simulink model "PCProject3"  (R2024a)
settings: Solver=VariableStepAuto  StartTime=0.0  StopTime=50.0  RelTol=1e-3
(part 1 of 7)
settings Model: Creator=User  LastModifiedBy=User

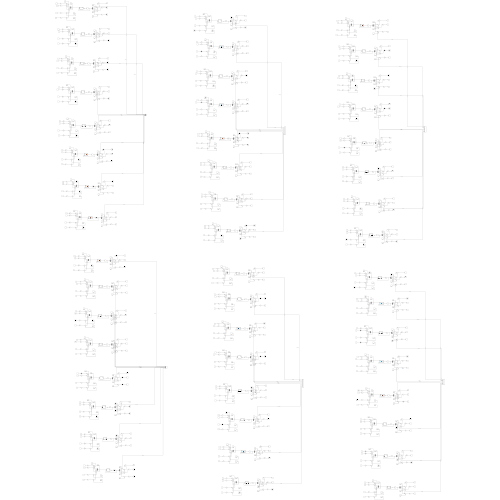
[thumbnail: Simulink's stored preview of the top-level diagram]
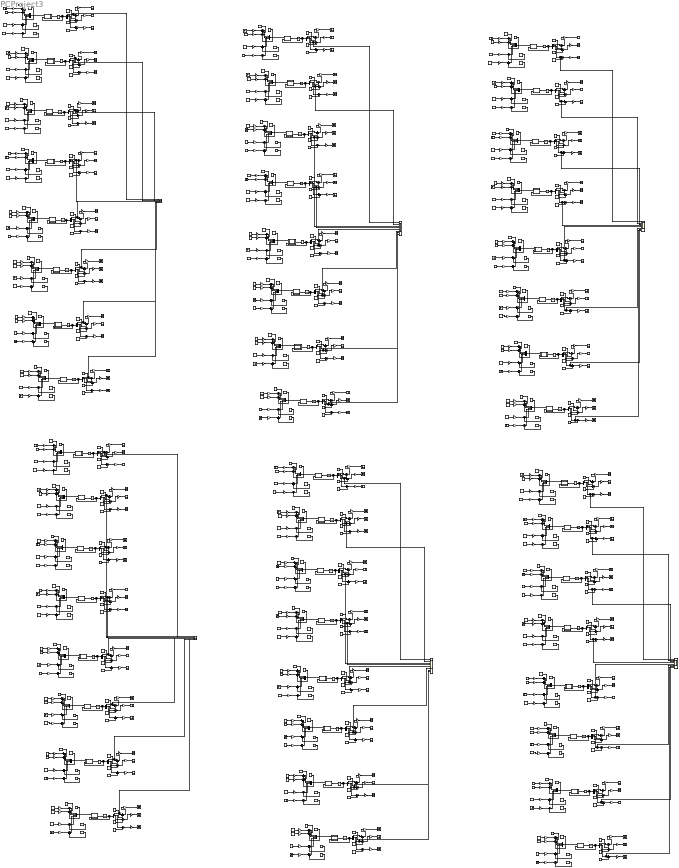
== system PCProject3 ==
  Bss{,1..47} (48 alike) : Constant  Value=9.44585785232475
  Constant{1..144} (144 alike) : Constant  Value=0
  Demux{,1..47} (48 alike) : Demux  Outputs=7
  F0ss{,1..47} (48 alike) : Constant  Value=100
  F_PUss{,1..47} (48 alike) : Constant  Value=25
  F_css{,1..47} (48 alike) : Constant  Value=500
  Gain{,7,14,21,28,35,42,49,56,62,70,77,85,93,100,109,112,118,126,133,141,149,156,165,168,171,180,184,190,199,207,214,216,224,232,242,250,257,265,273,280,288,295,303..304,311,320,329} (48 alike) : Gain  Gain=142.9/100
  Gain{1,8,15,22,29,36,43,50,57,63,71,78,86,94,102,110,113,119,127,134,142,150,158,166,169,173,182,185,191,200,208,217,225..226,234,243,251,258,266,274,282,289,296,305,312,314,321,330} (48 alike) : Gain  Gain=500/100
  Gain{3,10,17,24,31,38,45,52,58,65,73,79,81,88,96,104,114,121,129,135,137,144,152,160,170,175,186,194,202,209,211,219,228,237,245,253,259,261,268,276,284,290,298,307,313,316,323,332} (48 alike) : Gain  Gain=100/100
  Gain{5,12,19,26,33,40,46,54,60,67,75,83,91,98,101,106,116,123,131,139,147,154,157,162,172,177,188,192,196,205,213,222,230,233,239,247,255,263,271,278,281,286,293,300,309,318,327,334} (48 alike) : Gain  Gain=100/61.6246329506498
  Gain{2,9,16,23,30,37,44,51,64,68,72,80,87,95,103,111,120,124,128,136,143,151,159,167,174,183,193,197,201,210,218,227,235..236,244,248,252,260,267,275,283,297,301,306,315,322,325,331} (48 alike) : Gain  Gain=25/100
  Gain{4,11,18,25,32,39,53,59,66,74,82,89..90,97,105,115,122,130,138,145..146,153,161,176,181,187,195,204,212,220..221,229,238,246,254,262,269..270,277,285,291,299,308,317,324,326,333,336} (48 alike) : Gain  Gain=100/21.5066564396397
  Gain{6,13,20,27,34,41,47,55,61,69,76,84,92,99,107..108,117,125,132,140,148,155,163..164,178..179,189,198,203,206,215,223,231,240..241,249,256,264,272,279,287,292,294,302,310,319,328,335} (48 alike) : Gain  Gain=100/9.44585785232475
  Integrator : Integrator  InitialCondition=|
      | [21.5066564396397
      | 61.6246329506498
      | 9.44585785232475
      | 2.44473177554800
      | 0.491745288474893
      | 3.01943696537133
      | 2.73422289591667]
  Integrator1 : Integrator  InitialCondition=|
      | [21.5066564396397
      | 61.6246329506498
      | 9.44585785232475
      | 2.44473177554800
      | 0.491745288474893
      | 3.01943696537133
      | 2.73422289591667]
  Integrator10 : Integrator  InitialCondition=|
      | [21.5066564396397
      | 61.6246329506498
      | 9.44585785232475
      | 2.44473177554800
      | 0.491745288474893
      | 3.01943696537133
      | 2.73422289591667]
  Integrator11 : Integrator  InitialCondition=|
      | [21.5066564396397
      | 61.6246329506498
      | 9.44585785232475
      | 2.44473177554800
      | 0.491745288474893
      | 3.01943696537133
      | 2.73422289591667]
  Integrator12 : Integrator  InitialCondition=|
      | [21.5066564396397
      | 61.6246329506498
      | 9.44585785232475
      | 2.44473177554800
      | 0.491745288474893
      | 3.01943696537133
      | 2.73422289591667]
  Integrator13 : Integrator  InitialCondition=|
      | [21.5066564396397
      | 61.6246329506498
      | 9.44585785232475
      | 2.44473177554800
      | 0.491745288474893
      | 3.01943696537133
      | 2.73422289591667]
  Integrator14 : Integrator  InitialCondition=|
      | [21.5066564396397
      | 61.6246329506498
      | 9.44585785232475
      | 2.44473177554800
      | 0.491745288474893
      | 3.01943696537133
      | 2.73422289591667]
  Integrator15 : Integrator  InitialCondition=|
      | [21.5066564396397
      | 61.6246329506498
      | 9.44585785232475
      | 2.44473177554800
      | 0.491745288474893
      | 3.01943696537133
      | 2.73422289591667]
  Integrator16 : Integrator  InitialCondition=|
      | [21.5066564396397
      | 61.6246329506498
      | 9.44585785232475
      | 2.44473177554800
      | 0.491745288474893
      | 3.01943696537133
      | 2.73422289591667]
  Integrator17 : Integrator  InitialCondition=|
      | [21.5066564396397
      | 61.6246329506498
      | 9.44585785232475
      | 2.44473177554800
      | 0.491745288474893
      | 3.01943696537133
      | 2.73422289591667]
  Integrator18 : Integrator  InitialCondition=|
      | [21.5066564396397
      | 61.6246329506498
      | 9.44585785232475
      | 2.44473177554800
      | 0.491745288474893
      | 3.01943696537133
      | 2.73422289591667]
  Integrator19 : Integrator  InitialCondition=|
      | [21.5066564396397
      | 61.6246329506498
      | 9.44585785232475
      | 2.44473177554800
      | 0.491745288474893
      | 3.01943696537133
      | 2.73422289591667]
  Integrator2 : Integrator  InitialCondition=|
      | [21.5066564396397
      | 61.6246329506498
      | 9.44585785232475
      | 2.44473177554800
      | 0.491745288474893
      | 3.01943696537133
      | 2.73422289591667]
  Integrator20 : Integrator  InitialCondition=|
      | [21.5066564396397
      | 61.6246329506498
      | 9.44585785232475
      | 2.44473177554800
      | 0.491745288474893
      | 3.01943696537133
      | 2.73422289591667]
  Integrator21 : Integrator  InitialCondition=|
      | [21.5066564396397
      | 61.6246329506498
      | 9.44585785232475
      | 2.44473177554800
      | 0.491745288474893
      | 3.01943696537133
      | 2.73422289591667]
  Integrator22 : Integrator  InitialCondition=|
      | [21.5066564396397
      | 61.6246329506498
      | 9.44585785232475
      | 2.44473177554800
      | 0.491745288474893
      | 3.01943696537133
      | 2.73422289591667]
  Integrator23 : Integrator  InitialCondition=|
      | [21.5066564396397
      | 61.6246329506498
      | 9.44585785232475
      | 2.44473177554800
      | 0.491745288474893
      | 3.01943696537133
      | 2.73422289591667]
  Integrator24 : Integrator  InitialCondition=|
      | [21.5066564396397
      | 61.6246329506498
      | 9.44585785232475
      | 2.44473177554800
      | 0.491745288474893
      | 3.01943696537133
      | 2.73422289591667]
  Integrator25 : Integrator  InitialCondition=|
      | [21.5066564396397
      | 61.6246329506498
      | 9.44585785232475
      | 2.44473177554800
      | 0.491745288474893
      | 3.01943696537133
      | 2.73422289591667]
  Integrator26 : Integrator  InitialCondition=|
      | [21.5066564396397
      | 61.6246329506498
      | 9.44585785232475
      | 2.44473177554800
      | 0.491745288474893
      | 3.01943696537133
      | 2.73422289591667]
  Integrator27 : Integrator  InitialCondition=|
      | [21.5066564396397
      | 61.6246329506498
      | 9.44585785232475
      | 2.44473177554800
      | 0.491745288474893
      | 3.01943696537133
      | 2.73422289591667]
  Integrator28 : Integrator  InitialCondition=|
      | [21.5066564396397
      | 61.6246329506498
      | 9.44585785232475
      | 2.44473177554800
      | 0.491745288474893
      | 3.01943696537133
      | 2.73422289591667]
  Integrator29 : Integrator  InitialCondition=|
      | [21.5066564396397
      | 61.6246329506498
      | 9.44585785232475
      | 2.44473177554800
      | 0.491745288474893
      | 3.01943696537133
      | 2.73422289591667]
  Integrator3 : Integrator  InitialCondition=|
      | [21.5066564396397
      | 61.6246329506498
      | 9.44585785232475
      | 2.44473177554800
      | 0.491745288474893
      | 3.01943696537133
      | 2.73422289591667]
  Integrator30 : Integrator  InitialCondition=|
      | [21.5066564396397
      | 61.6246329506498
      | 9.44585785232475
      | 2.44473177554800
      | 0.491745288474893
      | 3.01943696537133
      | 2.73422289591667]
  Integrator31 : Integrator  InitialCondition=|
      | [21.5066564396397
      | 61.6246329506498
      | 9.44585785232475
      | 2.44473177554800
      | 0.491745288474893
      | 3.01943696537133
      | 2.73422289591667]
  Integrator32 : Integrator  InitialCondition=|
      | [21.5066564396397
      | 61.6246329506498
      | 9.44585785232475
      | 2.44473177554800
      | 0.491745288474893
      | 3.01943696537133
      | 2.73422289591667]
  Integrator33 : Integrator  InitialCondition=|
      | [21.5066564396397
      | 61.6246329506498
      | 9.44585785232475
      | 2.44473177554800
      | 0.491745288474893
      | 3.01943696537133
      | 2.73422289591667]
  Integrator34 : Integrator  InitialCondition=|
      | [21.5066564396397
      | 61.6246329506498
      | 9.44585785232475
      | 2.44473177554800
      | 0.491745288474893
      | 3.01943696537133
      | 2.73422289591667]
  Integrator35 : Integrator  InitialCondition=|
      | [21.5066564396397
      | 61.6246329506498
      | 9.44585785232475
      | 2.44473177554800
      | 0.491745288474893
      | 3.01943696537133
      | 2.73422289591667]
  Integrator36 : Integrator  InitialCondition=|
      | [21.5066564396397
      | 61.6246329506498
      | 9.44585785232475
      | 2.44473177554800
      | 0.491745288474893
      | 3.01943696537133
      | 2.73422289591667]
  Integrator37 : Integrator  InitialCondition=|
      | [21.5066564396397
      | 61.6246329506498
      | 9.44585785232475
      | 2.44473177554800
      | 0.491745288474893
      | 3.01943696537133
      | 2.73422289591667]
  Integrator38 : Integrator  InitialCondition=|
      | [21.5066564396397
      | 61.6246329506498
      | 9.44585785232475
      | 2.44473177554800
      | 0.491745288474893
      | 3.01943696537133
      | 2.73422289591667]
  Integrator39 : Integrator  InitialCondition=|
      | [21.5066564396397
      | 61.6246329506498
      | 9.44585785232475
      | 2.44473177554800
      | 0.491745288474893
      | 3.01943696537133
      | 2.73422289591667]
  Integrator4 : Integrator  InitialCondition=|
      | [21.5066564396397
      | 61.6246329506498
      | 9.44585785232475
      | 2.44473177554800
      | 0.491745288474893
      | 3.01943696537133
      | 2.73422289591667]
  Integrator40 : Integrator  InitialCondition=|
      | [21.5066564396397
      | 61.6246329506498
      | 9.44585785232475
      | 2.44473177554800
      | 0.491745288474893
      | 3.01943696537133
      | 2.73422289591667]
  Integrator41 : Integrator  InitialCondition=|
      | [21.5066564396397
      | 61.6246329506498
      | 9.44585785232475
      | 2.44473177554800
      | 0.491745288474893
      | 3.01943696537133
      | 2.73422289591667]
  Integrator42 : Integrator  InitialCondition=|
      | [21.5066564396397
      | 61.6246329506498
      | 9.44585785232475
      | 2.44473177554800
      | 0.491745288474893
      | 3.01943696537133
      | 2.73422289591667]
  Integrator43 : Integrator  InitialCondition=|
      | [21.5066564396397
      | 61.6246329506498
      | 9.44585785232475
      | 2.44473177554800
      | 0.491745288474893
      | 3.01943696537133
      | 2.73422289591667]
  Integrator44 : Integrator  InitialCondition=|
      | [21.5066564396397
      | 61.6246329506498
      | 9.44585785232475
      | 2.44473177554800
      | 0.491745288474893
      | 3.01943696537133
      | 2.73422289591667]
  Integrator45 : Integrator  InitialCondition=|
      | [21.5066564396397
      | 61.6246329506498
      | 9.44585785232475
      | 2.44473177554800
      | 0.491745288474893
      | 3.01943696537133
      | 2.73422289591667]
  Integrator46 : Integrator  InitialCondition=|
      | [21.5066564396397
      | 61.6246329506498
      | 9.44585785232475
      | 2.44473177554800
      | 0.491745288474893
      | 3.01943696537133
      | 2.73422289591667]
  Integrator47 : Integrator  InitialCondition=|
      | [21.5066564396397
      | 61.6246329506498
      | 9.44585785232475
      | 2.44473177554800
      | 0.491745288474893
      | 3.01943696537133
      | 2.73422289591667]
  Integrator5 : Integrator  InitialCondition=|
      | [21.5066564396397
      | 61.6246329506498
      | 9.44585785232475
      | 2.44473177554800
      | 0.491745288474893
      | 3.01943696537133
      | 2.73422289591667]
  Integrator6 : Integrator  InitialCondition=|
      | [21.5066564396397
      | 61.6246329506498
      | 9.44585785232475
      | 2.44473177554800
      | 0.491745288474893
      | 3.01943696537133
      | 2.73422289591667]
  Integrator7 : Integrator  InitialCondition=|
      | [21.5066564396397
      | 61.6246329506498
      | 9.44585785232475
      | 2.44473177554800
      | 0.491745288474893
      | 3.01943696537133
      | 2.73422289591667]
  Integrator8 : Integrator  InitialCondition=|
      | [21.5066564396397
      | 61.6246329506498
      | 9.44585785232475
      | 2.44473177554800
      | 0.491745288474893
      | 3.01943696537133
      | 2.73422289591667]
  Integrator9 : Integrator  InitialCondition=|
      | [21.5066564396397
      | 61.6246329506498
      | 9.44585785232475
      | 2.44473177554800
      | 0.491745288474893
      | 3.01943696537133
      | 2.73422289591667]
  MATLAB Function : MATLAB Function  TreatAsAtomicUnit=on
  MATLAB Function1 : MATLAB Function  TreatAsAtomicUnit=on
  MATLAB Function10 : MATLAB Function  TreatAsAtomicUnit=on
  MATLAB Function11 : MATLAB Function  TreatAsAtomicUnit=on
  MATLAB Function12 : MATLAB Function  TreatAsAtomicUnit=on
  MATLAB Function13 : MATLAB Function  TreatAsAtomicUnit=on
  MATLAB Function14 : MATLAB Function  TreatAsAtomicUnit=on
  MATLAB Function15 : MATLAB Function  TreatAsAtomicUnit=on
  MATLAB Function16 : MATLAB Function  TreatAsAtomicUnit=on
  MATLAB Function17 : MATLAB Function  TreatAsAtomicUnit=on
  MATLAB Function18 : MATLAB Function  TreatAsAtomicUnit=on
  MATLAB Function19 : MATLAB Function  TreatAsAtomicUnit=on
  MATLAB Function2 : MATLAB Function  TreatAsAtomicUnit=on
  MATLAB Function20 : MATLAB Function  TreatAsAtomicUnit=on
  MATLAB Function21 : MATLAB Function  TreatAsAtomicUnit=on
  MATLAB Function22 : MATLAB Function  TreatAsAtomicUnit=on
  MATLAB Function23 : MATLAB Function  TreatAsAtomicUnit=on
  MATLAB Function24 : MATLAB Function  TreatAsAtomicUnit=on
  MATLAB Function25 : MATLAB Function  TreatAsAtomicUnit=on
  MATLAB Function26 : MATLAB Function  TreatAsAtomicUnit=on
  MATLAB Function27 : MATLAB Function  TreatAsAtomicUnit=on
  MATLAB Function28 : MATLAB Function  TreatAsAtomicUnit=on
  MATLAB Function29 : MATLAB Function  TreatAsAtomicUnit=on
  MATLAB Function3 : MATLAB Function  TreatAsAtomicUnit=on
  MATLAB Function30 : MATLAB Function  TreatAsAtomicUnit=on
  MATLAB Function31 : MATLAB Function  TreatAsAtomicUnit=on
  MATLAB Function32 : MATLAB Function  TreatAsAtomicUnit=on
  MATLAB Function33 : MATLAB Function  TreatAsAtomicUnit=on
  MATLAB Function34 : MATLAB Function  TreatAsAtomicUnit=on
  MATLAB Function35 : MATLAB Function  TreatAsAtomicUnit=on
  MATLAB Function36 : MATLAB Function  TreatAsAtomicUnit=on
  MATLAB Function37 : MATLAB Function  TreatAsAtomicUnit=on
  MATLAB Function38 : MATLAB Function  TreatAsAtomicUnit=on
  MATLAB Function39 : MATLAB Function  TreatAsAtomicUnit=on
  MATLAB Function4 : MATLAB Function  TreatAsAtomicUnit=on
  MATLAB Function40 : MATLAB Function  TreatAsAtomicUnit=on
  MATLAB Function41 : MATLAB Function  TreatAsAtomicUnit=on
  MATLAB Function42 : MATLAB Function  TreatAsAtomicUnit=on
  MATLAB Function43 : MATLAB Function  TreatAsAtomicUnit=on
  MATLAB Function44 : MATLAB Function  TreatAsAtomicUnit=on
  MATLAB Function45 : MATLAB Function  TreatAsAtomicUnit=on
  MATLAB Function46 : MATLAB Function  TreatAsAtomicUnit=on
  MATLAB Function47 : MATLAB Function  TreatAsAtomicUnit=on
  MATLAB Function5 : MATLAB Function  TreatAsAtomicUnit=on
  MATLAB Function6 : MATLAB Function  TreatAsAtomicUnit=on
  MATLAB Function7 : MATLAB Function  TreatAsAtomicUnit=on
  MATLAB Function8 : MATLAB Function  TreatAsAtomicUnit=on
  MATLAB Function9 : MATLAB Function  TreatAsAtomicUnit=on
  Mux{,1..47} (48 alike) : Mux
  S0ss{,1..47} (48 alike) : Constant  Value=142.9
  Scope{,1..2,4..14,16..63,65..74,76..104,106..125,127..149} (144 alike) : Scope
  Scope{3,64,105,150..152} (6 alike) : Scope  NumInputPorts=8
  Sss{,1..47} (48 alike) : Constant  Value=61.6246329506498
  Step{,2,4..5,8,10,12..13,16,18,20..21} (12 alike) : Step  After=5  SampleTime=0
  Step{1,3,6..7,9,11,14..15,17,19,22..23} (12 alike) : Step  After=-5  SampleTime=0
  Step{24,26,28..29,32,34,36..38,42..43,46} (12 alike) : Step  After=30  SampleTime=0
  Step{25,27,30..31,33,35,39..41,44..45,47} (12 alike) : Step  After=-30  SampleTime=0
  Sum{,1..3,7..10,14..17,21..24,28..31,35..38,42..45,49..52,56..58,62..65,68,70..73,77..81,85..88,93..96,100,102..104,109..114,118..121,124,126..129,133..137,141..144,149..152,156,158..160,165..171,173..175,180,182..186,190..191,193..194,197,199..202,207..211,214,216..219,224..228,232,234..237,242..245,248,250..253,257..261,265..268,273..276,280,282..284,288..290,295..298,301,303..307,311..316,320..323,325,329..332} (192 alike) : Sum  Inputs=|++
  Sum{4..6,11..13,18..20,25..27,32..34,39..41,46..48,53..55,59..61,66..67,69,74..76,82..84,89..92,97..99,101,105..108,115..117,122..123,125,130..132,138..140,145..148,153..155,157,161..164,172,176..179,181,187..189,192,195..196,198,203..206,212..213,215,220..223,229..231,233,238..241,246..247,249,254..256,262..264,269..272,277..279,281,285..287,291..294,299..300,302,308..310,317..319,324,326..328,333..335} (144 alike) : Sum  Inputs=|+-
  Xss{,1..47} (48 alike) : Constant  Value=21.5066564396397
  wires:
  Gain2/1 -> Sum2/1
  Step/1 -> Gain/1
  Gain6/1 -> Scope2/1
  Sss/1 -> Sum5/2
  Gain3/1 -> Sum3/1
  Xss/1 -> Sum4/2
  Sum6/1 -> Gain6/1
  F0ss/1 -> Sum3/2
  F_PUss/1 -> Sum2/2
  Sum4/1 -> Gain4/1
  Constant1/1 -> Gain2/1
  Constant2/1 -> Gain1/1
  Bss/1 -> Sum6/2
  Sum5/1 -> Gain5/1
  Integrator/1 -> MATLAB Function/2(x), Demux/1  "x"
  S0ss/1 -> Sum/2
  Gain5/1 -> Scope1/1
  MATLAB Function/1(dxdt) -> Integrator/1  "dxdt"
  Gain4/1 -> Scope/1
  Constant4/1 -> Gain3/1
  Gain1/1 -> Sum1/1
  Mux/1 -> MATLAB Function/1(u)  "u"
  Gain/1 -> Sum/1
  F_css/1 -> Sum1/2
  Sum3/1 -> Mux/1
  Sum2/1 -> Mux/2
  Sum1/1 -> Mux/3
  Sum/1 -> Mux/4
  Demux/1 -> Sum4/1, Scope3/7  "-5% Fc"
  Demux/2 -> Sum5/1
  Demux/3 -> Sum6/1
  Step1/1 -> Gain7/1
  Xss1/1 -> Sum11/2
  MATLAB Function1/1(dxdt) -> Integrator1/1  "dxdt"
  Sum7/1 -> Mux1/4
  Demux1/3 -> Sum13/1
  Demux1/2 -> Sum12/1
  Sum13/1 -> Gain13/1
  Sum12/1 -> Gain12/1
  Constant3/1 -> Gain9/1
  Constant5/1 -> Gain8/1
  Gain9/1 -> Sum9/1
  Gain12/1 -> Scope7/1
  Integrator1/1 -> MATLAB Function1/2(x), Demux1/1  "x"
  Sum8/1 -> Mux1/3
  Gain8/1 -> Sum8/1
  Bss1/1 -> Sum13/2
  Demux1/1 -> Scope3/8, Sum11/1  "-5% S0"
  Sum9/1 -> Mux1/2
  Sum10/1 -> Mux1/1
  F_css1/1 -> Sum8/2
  Mux1/1 -> MATLAB Function1/1(u)  "u"
  Constant6/1 -> Gain10/1
  Gain7/1 -> Sum7/1
  F_PUss1/1 -> Sum9/2
  Gain11/1 -> Scope6/1
  Sum11/1 -> Gain11/1
  Gain13/1 -> Scope8/1
  Sss1/1 -> Sum12/2
  Gain10/1 -> Sum10/1
  F0ss1/1 -> Sum10/2
  S0ss1/1 -> Sum7/2
  Xss2/1 -> Sum18/2
  MATLAB Function2/1(dxdt) -> Integrator2/1  "dxdt"
  Sum14/1 -> Mux2/4
  Demux2/3 -> Sum20/1
  Demux2/2 -> Sum19/1
  Sum20/1 -> Gain20/1
  Sum19/1 -> Gain19/1
  Constant8/1 -> Gain15/1
  Gain16/1 -> Sum16/1
  Gain19/1 -> Scope12/1
  Integrator2/1 -> MATLAB Function2/2(x), Demux2/1  "x"
  Sum15/1 -> Mux2/3
  Gain15/1 -> Sum15/1
  Bss2/1 -> Sum20/2
  Demux2/1 -> Scope3/3, Sum18/1  "+5% Fc"
  Sum16/1 -> Mux2/2
  Sum17/1 -> Mux2/1
  F_css2/1 -> Sum15/2
  Mux2/1 -> MATLAB Function2/1(u)  "u"
  Constant9/1 -> Gain17/1
  Gain14/1 -> Sum14/1
  F_PUss2/1 -> Sum16/2
  Gain18/1 -> Scope11/1
  Sum18/1 -> Gain18/1
  Gain20/1 -> Scope13/1
  Sss2/1 -> Sum19/2
  Gain17/1 -> Sum17/1
  F0ss2/1 -> Sum17/2
  S0ss2/1 -> Sum14/2
  Xss3/1 -> Sum25/2
  MATLAB Function3/1(dxdt) -> Integrator3/1  "dxdt"
  Sum21/1 -> Mux3/4
  Demux3/3 -> Sum27/1
  Demux3/2 -> Sum26/1
  Sum27/1 -> Gain27/1
  Sum26/1 -> Gain26/1
  Constant11/1 -> Gain22/1
  Gain23/1 -> Sum23/1
  Gain26/1 -> Scope17/1
  Integrator3/1 -> MATLAB Function3/2(x), Demux3/1  "x"
  Sum22/1 -> Mux3/3
  Gain22/1 -> Sum22/1
  Bss3/1 -> Sum27/2
  Demux3/1 -> Scope3/4, Sum25/1  "+5% S0"
  Sum23/1 -> Mux3/2
  Sum24/1 -> Mux3/1
  F_css3/1 -> Sum22/2
  Mux3/1 -> MATLAB Function3/1(u)  "u"
  Constant12/1 -> Gain24/1
  Gain21/1 -> Sum21/1
  F_PUss3/1 -> Sum23/2
  Gain25/1 -> Scope16/1
  Sum25/1 -> Gain25/1
  Gain27/1 -> Scope18/1
  Sss3/1 -> Sum26/2
  Gain24/1 -> Sum24/1
  F0ss3/1 -> Sum24/2
  S0ss3/1 -> Sum21/2
  Xss4/1 -> Sum32/2
  MATLAB Function4/1(dxdt) -> Integrator4/1  "dxdt"
  Sum28/1 -> Mux4/4
  Demux4/3 -> Sum34/1
  Demux4/2 -> Sum33/1
  Sum34/1 -> Gain34/1
  Sum33/1 -> Gain33/1
  Constant13/1 -> Gain30/1
  Gain30/1 -> Sum30/1
  Gain33/1 -> Scope22/1
  Integrator4/1 -> MATLAB Function4/2(x), Demux4/1  "x"
  Sum29/1 -> Mux4/3
  Gain29/1 -> Sum29/1
  Bss4/1 -> Sum34/2
  Demux4/1 -> Scope3/5, Sum32/1  "-5% F0"
  Sum30/1 -> Mux4/2
  Sum31/1 -> Mux4/1
  F_css4/1 -> Sum29/2
  Mux4/1 -> MATLAB Function4/1(u)  "u"
  Constant15/1 -> Gain31/1
  Gain28/1 -> Sum28/1
  F_PUss4/1 -> Sum30/2
  Gain32/1 -> Scope21/1
  Sum32/1 -> Gain32/1
  Gain34/1 -> Scope23/1
  Sss4/1 -> Sum33/2
  Gain31/1 -> Sum31/1
  F0ss4/1 -> Sum31/2
  S0ss4/1 -> Sum28/2
  Xss5/1 -> Sum39/2
  MATLAB Function5/1(dxdt) -> Integrator5/1  "dxdt"
  Sum35/1 -> Mux5/4
  Demux5/3 -> Sum41/1
  Demux5/2 -> Sum40/1
  Sum41/1 -> Gain41/1
  Sum40/1 -> Gain40/1
  Constant16/1 -> Gain37/1
  Constant17/1 -> Gain36/1
  Gain37/1 -> Sum37/1
  Gain40/1 -> Scope27/1
  Integrator5/1 -> MATLAB Function5/2(x), Demux5/1  "x"
  Sum36/1 -> Mux5/3
  Gain36/1 -> Sum36/1
  Bss5/1 -> Sum41/2
  Sum37/1 -> Mux5/2
  Sum38/1 -> Mux5/1
  F_css5/1 -> Sum36/2
  Mux5/1 -> MATLAB Function5/1(u)  "u"
  Gain35/1 -> Sum35/1
  F_PUss5/1 -> Sum37/2
  Gain39/1 -> Scope26/1
  Sum39/1 -> Gain39/1
  Gain41/1 -> Scope28/1
  Sss5/1 -> Sum40/2
  Gain38/1 -> Sum38/1
  F0ss5/1 -> Sum38/2
  S0ss5/1 -> Sum35/2
  Xss6/1 -> Sum46/2
  MATLAB Function6/1(dxdt) -> Integrator6/1  "dxdt"
  Sum42/1 -> Mux6/4
  Demux6/3 -> Sum48/1
  Demux6/2 -> Sum47/1
  Sum48/1 -> Gain47/1
  Sum47/1 -> Gain46/1
  Constant19/1 -> Gain44/1
  Constant20/1 -> Gain43/1
  Gain44/1 -> Sum44/1
  Gain46/1 -> Scope32/1
  Integrator6/1 -> MATLAB Function6/2(x), Demux6/1  "x"
  Sum43/1 -> Mux6/3
  Gain43/1 -> Sum43/1
  Bss6/1 -> Sum48/2
  Sum44/1 -> Mux6/2
  Sum45/1 -> Mux6/1
  F_css6/1 -> Sum43/2
  Mux6/1 -> MATLAB Function6/1(u)  "u"
  Gain42/1 -> Sum42/1
  F_PUss6/1 -> Sum44/2
  Gain336/1 -> Scope31/1
  Sum46/1 -> Gain336/1
  Gain47/1 -> Scope33/1
  Sss6/1 -> Sum47/2
  Gain45/1 -> Sum45/1
  F0ss6/1 -> Sum45/2
  S0ss6/1 -> Sum42/2
  Xss7/1 -> Sum53/2
  MATLAB Function7/1(dxdt) -> Integrator7/1  "dxdt"
  Sum49/1 -> Mux7/4
  Demux7/3 -> Sum55/1
  Demux7/2 -> Sum54/1
  Sum55/1 -> Gain55/1
  Sum54/1 -> Gain54/1
  Constant22/1 -> Gain51/1
  Gain51/1 -> Sum51/1
  Gain54/1 -> Scope37/1
  Integrator7/1 -> MATLAB Function7/2(x), Demux7/1  "x"
  Sum50/1 -> Mux7/3
  Gain50/1 -> Sum50/1
  Bss7/1 -> Sum55/2
  Demux7/1 -> Sum53/1, Scope3/6  "-5% F_PU"
  Sum51/1 -> Mux7/2
  Sum52/1 -> Mux7/1
  F_css7/1 -> Sum50/2
  Mux7/1 -> MATLAB Function7/1(u)  "u"
  Constant24/1 -> Gain52/1
  Gain49/1 -> Sum49/1
  F_PUss7/1 -> Sum51/2
  Gain53/1 -> Scope36/1
  Sum53/1 -> Gain53/1
  Gain55/1 -> Scope38/1
  Sss7/1 -> Sum54/2
  Gain52/1 -> Sum52/1
  F0ss7/1 -> Sum52/2
  S0ss7/1 -> Sum49/2
  Constant18/1 -> Gain35/1
  Step5/1 -> Gain38/1
  Constant21/1 -> Gain42/1
  Step6/1 -> Gain45/1
  Constant7/1 -> Gain14/1
  Step2/1 -> Gain16/1
  Constant10/1 -> Gain21/1
  Step3/1 -> Gain23/1
  Constant14/1 -> Gain28/1
  Step4/1 -> Gain29/1
  Constant23/1 -> Gain49/1
  Step7/1 -> Gain50/1
  Gain70/1 -> Sum70/1
  Constant30/1 -> Gain77/1
  Demux11/2 -> Scope64/4, Sum75/1  "+5% S0"
  Sum78/1 -> Mux12/3
  Mux9/1 -> MATLAB Function9/1(u)  "u"
  Sum111/1 -> Mux9/2
  Sum88/1 -> Mux13/1
  Demux12/1 -> Sum82/1
  F0ss9/1 -> Sum58/2
  Gain106/1 -> Scope72/1
  Sum104/1 -> Mux15/1
  F_css9/1 -> Sum110/2
  Constant39/1 -> Gain103/1
  MATLAB Function12/1(dxdt) -> Integrator12/1  "dxdt"
  Mux10/1 -> MATLAB Function10/1(u)  "u"
  Sum66/1 -> Gain66/1
  Sum69/1 -> Gain69/1
  Step14/1 -> Gain96/1
  Constant40/1 -> Gain100/1
  Sum106/1 -> Gain106/1
  Mux15/1 -> MATLAB Function15/1(u)  "u"
  F_PUss14/1 -> Sum95/2
  Demux14/2 -> Scope64/2, Sum98/1  "+5% F_PU"
  Demux14/1 -> Sum97/1
  S0ss9/1 -> Sum109/2
  Sss9/1 -> Sum60/2
  F0ss14/1 -> Sum96/2
  Bss8/1 -> Sum108/2
  Constant48/1 -> Gain65/1
  Constant38/1 -> Gain93/1
  Demux9/1 -> Sum59/1
  Mux8/1 -> MATLAB Function8/1(u)  "u"
  Gain99/1 -> Scope68/1
  Gain110/1 -> Sum110/1
  S0ss15/1 -> Sum100/2
  Gain81/1 -> Sum81/1
  Gain105/1 -> Scope71/1
  Step13/1 -> Gain88/1
  F_PUss15/1 -> Sum103/2
  Demux8/2 -> Scope64/7, Sum101/1  "-5% Fc"
  Demux10/3 -> Sum69/1
  Gain104/1 -> Sum104/1
  Demux15/1 -> Sum105/1
  Gain107/1 -> Scope73/1
  S0ss14/1 -> Sum93/2
  Xss15/1 -> Sum105/2
  Mux11/1 -> MATLAB Function11/1(u)  "u"
  Integrator15/1 -> MATLAB Function15/2(x), Demux15/1  "x"
  Constant29/1 -> Gain80/1
  Constant36/1 -> Gain57/1
  Step8/1 -> Gain56/1
  Bss15/1 -> Sum107/2
  Xss12/1 -> Sum82/2
  Gain97/1 -> Scope66/1
  F_css10/1 -> Sum63/2
  Sum96/1 -> Mux14/1
  Sum107/1 -> Gain107/1
  Gain77/1 -> Sum77/1
  Sum79/1 -> Mux8/1
  Xss14/1 -> Sum97/2
  Constant46/1 -> Gain62/1
  Constant33/1 -> Gain86/1
  Gain103/1 -> Sum103/1
  Gain101/1 -> Scope42/1
  Bss11/1 -> Sum76/2
  Sum102/1 -> Mux15/3
  S0ss8/1 -> Sum56/2
  F0ss8/1 -> Sum79/2
  Sum103/1 -> Mux15/2
  Gain61/1 -> Scope80/1
  F_css12/1 -> Sum78/2
  Sum65/1 -> Mux10/1
  Demux15/2 -> Scope64/6, Sum106/1  "-5% F_PU"
  Demux15/3 -> Sum107/1
  Sum73/1 -> Mux11/1
  Sum87/1 -> Mux13/2
  Gain98/1 -> Scope67/1
  Sum89/1 -> Gain89/1
  Sum58/1 -> Mux9/1
  F_css14/1 -> Sum94/2
  Sss12/1 -> Sum83/2
  Step11/1 -> Gain72/1
  Demux9/2 -> Scope64/8, Sum60/1  "-5% S0"
  Integrator12/1 -> MATLAB Function12/2(x), Demux12/1  "x"
  Sum70/1 -> Mux11/4
  Sum97/1 -> Gain97/1
  Sum93/1 -> Mux14/4
  Sss13/1 -> Sum91/2
  Sum94/1 -> Mux14/3
  Sum101/1 -> Gain101/1
  Sum59/1 -> Gain59/1
  Sum99/1 -> Gain99/1
  Bss14/1 -> Sum99/2
  Integrator14/1 -> MATLAB Function14/2(x), Demux14/1  "x"
  Gain92/1 -> Scope62/1
  Gain87/1 -> Sum87/1
  F_PUss8/1 -> Sum68/2
  Gain94/1 -> Sum94/1
  S0ss12/1 -> Sum77/2
  F0ss15/1 -> Sum104/2
  Gain82/1 -> Scope55/1
  Bss10/1 -> Sum69/2
  Gain89/1 -> Scope60/1
  Bss13/1 -> Sum92/2
  F0ss13/1 -> Sum88/2
  Constant27/1 -> Gain71/1
  F_PUss13/1 -> Sum87/2
  Constant42/1 -> Gain111/1
  Step12/1 -> Gain78/1
  F_css8/1 -> Sum57/2
  Gain86/1 -> Sum86/1
  Sum86/1 -> Mux13/3
  MATLAB Function11/1(dxdt) -> Integrator11/1  "dxdt"
  Mux13/1 -> MATLAB Function13/1(u)  "u"
  Integrator9/1 -> MATLAB Function9/2(x), Demux9/1  "x"
  Gain85/1 -> Sum85/1
  Integrator13/1 -> MATLAB Function13/2(x), Demux13/1  "x"
  Sum72/1 -> Mux11/2
  Gain91/1 -> Scope61/1
  Step9/1 -> Gain109/1
  Gain73/1 -> Sum73/1
  Sum84/1 -> Gain84/1
  Gain56/1 -> Sum56/1
  Mux12/1 -> MATLAB Function12/1(u)  "u"
  Gain58/1 -> Sum58/1
  Constant37/1 -> Gain94/1
  Xss13/1 -> Sum89/2
  Demux13/3 -> Sum92/1
  Integrator10/1 -> MATLAB Function10/2(x), Demux10/1  "x"
  Constant32/1 -> Gain87/1
  S0ss11/1 -> Sum70/2
  Gain76/1 -> Scope51/1
  F0ss12/1 -> Sum81/2
  Sum92/1 -> Gain92/1
  Demux13/2 -> Scope64/1, Sum91/1  "+5% F0"
  Sum80/1 -> Mux12/2
  Sum77/1 -> Mux12/4
  Sum82/1 -> Gain82/1
  Demux12/2 -> Scope64/5, Sum83/1  "-5% F0"
  Xss9/1 -> Sum59/2
  F_css15/1 -> Sum102/2
  Constant31/1 -> Gain81/1
  Sum81/1 -> Mux12/1
  Constant25/1 -> Gain68/1
  MATLAB Function14/1(dxdt) -> Integrator14/1  "dxdt"
  F_PUss12/1 -> Sum80/2
  Gain57/1 -> Sum57/1
  Demux12/3 -> Sum84/1
  Constant41/1 -> Gain104/1
  Sss15/1 -> Sum106/2
  Gain83/1 -> Scope56/1
  Gain84/1 -> Scope57/1
  Demux13/1 -> Sum89/1
  F0ss10/1 -> Sum65/2
  Gain80/1 -> Sum80/1
  Sum100/1 -> Mux15/4
  Gain71/1 -> Sum71/1
  Constant28/1 -> Gain73/1
  F_PUss11/1 -> Sum72/2
  Sum71/1 -> Mux11/3
  Sum110/1 -> Mux9/3
  Sum105/1 -> Gain105/1
  Gain74/1 -> Scope49/1
  MATLAB Function10/1(dxdt) -> Integrator10/1  "dxdt"
  MATLAB Function13/1(dxdt) -> Integrator13/1  "dxdt"
  F_css11/1 -> Sum71/2
  Step10/1 -> Gain64/1
  Sum75/1 -> Gain75/1
  Sum98/1 -> Gain98/1
  Gain69/1 -> Scope46/1
  Sum91/1 -> Gain91/1
  Constant45/1 -> Gain58/1
  Constant35/1 -> Gain95/1
  Gain66/1 -> Scope44/1
  MATLAB Function15/1(dxdt) -> Integrator15/1  "dxdt"
  Demux10/1 -> Sum66/1
  Sum108/1 -> Gain108/1
  Gain78/1 -> Sum78/1
  Sss11/1 -> Sum75/2
  Gain102/1 -> Sum102/1
  Gain65/1 -> Sum65/1
  Sum109/1 -> Mux9/4
  Gain96/1 -> Sum96/1
  Sum62/1 -> Mux10/4
  Gain100/1 -> Sum100/1
  Demux11/1 -> Sum74/1
  Sum85/1 -> Mux13/4
  Xss10/1 -> Sum66/2
  Gain67/1 -> Scope45/1
  Gain59/1 -> Scope78/1
  Sum74/1 -> Gain74/1
  Gain64/1 -> Sum64/1
  Demux14/3 -> Sum99/1
  Step15/1 -> Gain102/1
  Constant34/1 -> Gain85/1
  Demux10/2 -> Scope64/3, Sum67/1  "+5% Fc"
  Bss12/1 -> Sum84/2
  Gain63/1 -> Sum63/1
  Gain62/1 -> Sum62/1
  Gain111/1 -> Sum111/1
  Sss14/1 -> Sum98/2
  Constant44/1 -> Gain110/1
  Sum60/1 -> Gain60/1
  Sum61/1 -> Gain61/1
  Gain108/1 -> Scope53/1
  Constant47/1 -> Gain63/1
  Demux9/3 -> Sum61/1
  S0ss10/1 -> Sum62/2
  Integrator8/1 -> MATLAB Function8/2(x), Demux8/1  "x"
  F_css13/1 -> Sum86/2
  Constant43/1 -> Gain79/1
  Gain88/1 -> Sum88/1
  Gain109/1 -> Sum109/1
  Sum64/1 -> Mux10/2
  F0ss11/1 -> Sum73/2
  Sum63/1 -> Mux10/3
  Demux8/1 -> Sum90/1
  Gain90/1 -> Scope41/1
  F_PUss10/1 -> Sum64/2
  Demux8/3 -> Sum108/1
  Gain60/1 -> Scope79/1
  MATLAB Function9/1(dxdt) -> Integrator9/1  "dxdt"
  Integrator11/1 -> MATLAB Function11/2(x), Demux11/1  "x"
  Gain75/1 -> Scope50/1
  Gain72/1 -> Sum72/1
  S0ss13/1 -> Sum85/2
  Gain95/1 -> Sum95/1
  Sum68/1 -> Mux8/2
  Sss10/1 -> Sum67/2
  Sum90/1 -> Gain90/1
  Sum57/1 -> Mux8/3
  Gain68/1 -> Sum68/1
  MATLAB Function8/1(dxdt) -> Integrator8/1  "dxdt"
  Gain93/1 -> Sum93/1
  Sss8/1 -> Sum101/2
  Mux14/1 -> MATLAB Function14/1(u)  "u"
  Xss8/1 -> Sum90/2
  Sum83/1 -> Gain83/1
  Gain79/1 -> Sum79/1
  Sum95/1 -> Mux14/2
  Xss11/1 -> Sum74/2
  Bss9/1 -> Sum61/2
  Sum56/1 -> Mux8/4
  Demux11/3 -> Sum76/1
  Sum76/1 -> Gain76/1
  F_PUss9/1 -> Sum111/2
  Constant26/1 -> Gain70/1
  Gain126/1 -> Sum126/1
  Constant54/1 -> Gain133/1
  Demux19/2 -> Sum131/1
  Sum134/1 -> Mux20/3
  Mux17/1 -> MATLAB Function17/1(u)  "u"
  Sum167/1 -> Mux17/2
  Sum144/1 -> Mux21/1
  Demux20/1 -> Sum138/1
  F0ss17/1 -> Sum114/2
  Gain162/1 -> Scope113/1
  Sum160/1 -> Mux23/1
  F_css17/1 -> Sum166/2
  Constant63/1 -> Gain159/1
  MATLAB Function20/1(dxdt) -> Integrator20/1  "dxdt"
  Mux18/1 -> MATLAB Function18/1(u)  "u"
  Sum122/1 -> Gain122/1
  Sum125/1 -> Gain125/1
  Step22/1 -> Gain152/1
  Constant64/1 -> Gain156/1
  Sum162/1 -> Gain162/1
  Mux23/1 -> MATLAB Function23/1(u)  "u"
  F_PUss22/1 -> Sum151/2
  Demux22/2 -> Sum154/1
  Demux22/1 -> Sum153/1
  S0ss17/1 -> Sum165/2
  Sss17/1 -> Sum116/2
  F0ss22/1 -> Sum152/2
  Bss16/1 -> Sum164/2
  Constant72/1 -> Gain121/1
  Constant62/1 -> Gain149/1
  Demux17/1 -> Sum115/1
  Mux16/1 -> MATLAB Function16/1(u)  "u"
  Gain155/1 -> Scope109/1
  Gain166/1 -> Sum166/1
  S0ss23/1 -> Sum156/2
  Gain137/1 -> Sum137/1
  Gain161/1 -> Scope112/1
  Step21/1 -> Gain144/1
  F_PUss23/1 -> Sum159/2
  Demux16/2 -> Sum157/1
  Demux18/3 -> Scope105/3, Sum125/1  "+5% Fc"
  Gain160/1 -> Sum160/1
  Demux23/1 -> Sum161/1
  Gain163/1 -> Scope114/1
  S0ss22/1 -> Sum149/2
  Xss23/1 -> Sum161/2
  Mux19/1 -> MATLAB Function19/1(u)  "u"
  Integrator23/1 -> MATLAB Function23/2(x), Demux23/1  "x"
  Constant53/1 -> Gain136/1
  Constant60/1 -> Gain113/1
  Step16/1 -> Gain112/1
  Bss23/1 -> Sum163/2
  Xss20/1 -> Sum138/2
  Gain153/1 -> Scope107/1
  F_css18/1 -> Sum119/2
  Sum152/1 -> Mux22/1
  Sum163/1 -> Gain163/1
  Gain133/1 -> Sum133/1
  Sum135/1 -> Mux16/1
  Xss22/1 -> Sum153/2
  Constant70/1 -> Gain118/1
  Constant57/1 -> Gain142/1
  Gain159/1 -> Sum159/1
  Gain157/1 -> Scope83/1
  Bss19/1 -> Sum132/2
  Sum158/1 -> Mux23/3
  S0ss16/1 -> Sum112/2
  F0ss16/1 -> Sum135/2
  Sum159/1 -> Mux23/2
  Gain117/1 -> Scope121/1
  F_css20/1 -> Sum134/2
  Sum121/1 -> Mux18/1
  Demux23/2 -> Sum162/1
  Demux23/3 -> Scope105/6, Sum163/1  "-5% F_PU"
  Sum129/1 -> Mux19/1
  Sum143/1 -> Mux21/2
  Gain154/1 -> Scope108/1
  Sum145/1 -> Gain145/1
  Sum114/1 -> Mux17/1
  F_css22/1 -> Sum150/2
  Sss20/1 -> Sum139/2
  Step19/1 -> Gain128/1
  Demux17/2 -> Sum116/1
  Integrator20/1 -> MATLAB Function20/2(x), Demux20/1  "x"
  Sum126/1 -> Mux19/4
  Sum153/1 -> Gain153/1
  Sum149/1 -> Mux22/4
  Sss21/1 -> Sum147/2
  Sum150/1 -> Mux22/3
  Sum157/1 -> Gain157/1
  Sum115/1 -> Gain115/1
  Sum155/1 -> Gain155/1
  Bss22/1 -> Sum155/2
  Integrator22/1 -> MATLAB Function22/2(x), Demux22/1  "x"
  Gain148/1 -> Scope103/1
  Gain143/1 -> Sum143/1
  F_PUss16/1 -> Sum124/2
  Gain150/1 -> Sum150/1
  S0ss20/1 -> Sum133/2
  F0ss23/1 -> Sum160/2
  Gain138/1 -> Scope96/1
  Bss18/1 -> Sum125/2
  Gain145/1 -> Scope101/1
  Bss21/1 -> Sum148/2
  F0ss21/1 -> Sum144/2
  Constant51/1 -> Gain127/1
  F_PUss21/1 -> Sum143/2
  Constant66/1 -> Gain167/1
  Step20/1 -> Gain134/1
  F_css16/1 -> Sum113/2
  Gain142/1 -> Sum142/1
  Sum142/1 -> Mux21/3
  MATLAB Function19/1(dxdt) -> Integrator19/1  "dxdt"
  Mux21/1 -> MATLAB Function21/1(u)  "u"
  Integrator17/1 -> MATLAB Function17/2(x), Demux17/1  "x"
  Gain141/1 -> Sum141/1
  Integrator21/1 -> MATLAB Function21/2(x), Demux21/1  "x"
  Sum128/1 -> Mux19/2
  Gain147/1 -> Scope102/1
  Step17/1 -> Gain165/1
  Gain129/1 -> Sum129/1
  Sum140/1 -> Gain140/1
  Gain112/1 -> Sum112/1
  Mux20/1 -> MATLAB Function20/1(u)  "u"
  Gain114/1 -> Sum114/1
  Constant61/1 -> Gain150/1
  Xss21/1 -> Sum145/2
  Demux21/3 -> Scope105/1, Sum148/1  "+5% F0"
  Integrator18/1 -> MATLAB Function18/2(x), Demux18/1  "x"
  Constant56/1 -> Gain143/1
  S0ss19/1 -> Sum126/2
  Gain132/1 -> Scope92/1
  F0ss20/1 -> Sum137/2
  Sum148/1 -> Gain148/1
  Demux21/2 -> Sum147/1
  Sum136/1 -> Mux20/2
  Sum133/1 -> Mux20/4
  Sum138/1 -> Gain138/1
  Demux20/2 -> Sum139/1
  Xss17/1 -> Sum115/2
  F_css23/1 -> Sum158/2
  Constant55/1 -> Gain137/1
  Sum137/1 -> Mux20/1
  Constant49/1 -> Gain124/1
  MATLAB Function22/1(dxdt) -> Integrator22/1  "dxdt"
  F_PUss20/1 -> Sum136/2
  Gain113/1 -> Sum113/1
  Demux20/3 -> Scope105/5, Sum140/1  "-5% F0"
  Constant65/1 -> Gain160/1
  Sss23/1 -> Sum162/2
  Gain139/1 -> Scope97/1
  Gain140/1 -> Scope98/1
  Demux21/1 -> Sum145/1
  F0ss18/1 -> Sum121/2
  Gain136/1 -> Sum136/1
  Sum156/1 -> Mux23/4
  Gain127/1 -> Sum127/1
  Constant52/1 -> Gain129/1
  F_PUss19/1 -> Sum128/2
  Sum127/1 -> Mux19/3
  Sum166/1 -> Mux17/3
  Sum161/1 -> Gain161/1
  Gain130/1 -> Scope90/1
  MATLAB Function18/1(dxdt) -> Integrator18/1  "dxdt"
  MATLAB Function21/1(dxdt) -> Integrator21/1  "dxdt"
  F_css19/1 -> Sum127/2
  Step18/1 -> Gain120/1
  Sum131/1 -> Gain131/1
  Sum154/1 -> Gain154/1
  Gain125/1 -> Scope87/1
  Sum147/1 -> Gain147/1
  Constant69/1 -> Gain114/1
  Constant59/1 -> Gain151/1
  Gain122/1 -> Scope85/1
  MATLAB Function23/1(dxdt) -> Integrator23/1  "dxdt"
  Demux18/1 -> Sum122/1
  Sum164/1 -> Gain164/1
  Gain134/1 -> Sum134/1
  Sss19/1 -> Sum131/2
  Gain158/1 -> Sum158/1
  Gain121/1 -> Sum121/1
  Sum165/1 -> Mux17/4
  Gain152/1 -> Sum152/1
  Sum118/1 -> Mux18/4
  Gain156/1 -> Sum156/1
  Demux19/1 -> Sum130/1
  Sum141/1 -> Mux21/4
  Xss18/1 -> Sum122/2
  Gain123/1 -> Scope86/1
  Gain115/1 -> Scope119/1
  Sum130/1 -> Gain130/1
  Gain120/1 -> Sum120/1
  Demux22/3 -> Scope105/2, Sum155/1  "+5% F_PU"
  Step23/1 -> Gain158/1
  Constant58/1 -> Gain141/1
  Demux18/2 -> Sum123/1
  Bss20/1 -> Sum140/2
  Gain119/1 -> Sum119/1
  Gain118/1 -> Sum118/1
  Sum123/1 -> Gain123/1
  Gain167/1 -> Sum167/1
  Sss22/1 -> Sum154/2
  Constant68/1 -> Gain166/1
  Sum116/1 -> Gain116/1
  Sum117/1 -> Gain117/1
  Gain164/1 -> Scope94/1
  Constant71/1 -> Gain119/1
  Demux17/3 -> Scope105/8, Sum117/1  "-5% S0"
  S0ss18/1 -> Sum118/2
  Integrator16/1 -> MATLAB Function16/2(x), Demux16/1  "x"
  F_css21/1 -> Sum142/2
  Constant67/1 -> Gain135/1
  Gain144/1 -> Sum144/1
  Gain165/1 -> Sum165/1
  Sum120/1 -> Mux18/2
  F0ss19/1 -> Sum129/2
  Sum119/1 -> Mux18/3
  Demux16/1 -> Sum146/1
  Gain146/1 -> Scope82/1
  F_PUss18/1 -> Sum120/2
  Demux16/3 -> Scope105/7, Sum164/1  "-5% Fc"
  Gain116/1 -> Scope120/1
  MATLAB Function17/1(dxdt) -> Integrator17/1  "dxdt"
  Integrator19/1 -> MATLAB Function19/2(x), Demux19/1  "x"
  Gain131/1 -> Scope91/1
  Gain128/1 -> Sum128/1
  S0ss21/1 -> Sum141/2
  Gain151/1 -> Sum151/1
  Sum124/1 -> Mux16/2
  Sss18/1 -> Sum123/2
  Sum146/1 -> Gain146/1
  Sum113/1 -> Mux16/3
  Gain124/1 -> Sum124/1
  MATLAB Function16/1(dxdt) -> Integrator16/1  "dxdt"
  Gain149/1 -> Sum149/1
  Sss16/1 -> Sum157/2
  Mux22/1 -> MATLAB Function22/1(u)  "u"
  Xss16/1 -> Sum146/2
  Sum139/1 -> Gain139/1
  Gain135/1 -> Sum135/1
  Sum151/1 -> Mux22/2
  Xss19/1 -> Sum130/2
  Bss17/1 -> Sum117/2
  Sum112/1 -> Mux16/4
  Demux19/3 -> Scope105/4, Sum132/1  "+5% S0"
  Sum132/1 -> Gain132/1
  F_PUss17/1 -> Sum167/2
  Constant50/1 -> Gain126/1
  Sum67/1 -> Gain67/1
  Demux5/1 -> Scope3/1, Sum39/1  "+5% F0"
  Demux6/1 -> Scope3/2, Sum46/1  "+5% F_PU"
  Gain187/1 -> Scope35/1
  MATLAB Function38/1(dxdt) -> Integrator38/1  "dxdt"
  Bss37/1 -> Sum215/2
  Sum224/1 -> Mux39/4
  Demux35/1 -> Sum204/1
  Sss35/1 -> Sum205/2
  Sum223/1 -> Gain223/1
  Constant138/1 -> Gain186/1
  Demux33/2 -> Sum188/1
  Sum230/1 -> Gain230/1
  Demux38/1 -> Sum220/1
  Sum173/1 -> Mux31/3
  Gain210/1 -> Sum210/1
  Demux37/3 -> Scope150/5, Sum215/1  "-30% F0"
  MATLAB Function39/1(dxdt) -> Integrator39/1  "dxdt"
  F_PUss37/1 -> Sum210/2
  Xss33/1 -> Sum187/2
  Integrator47/1 -> MATLAB Function47/2(x), Demux47/1  "x"
  Demux41/2 -> Sum255/1
  Gain324/1 -> Scope123/1
  F_css24/1 -> Sum169/2
  Sum333/1 -> Gain333/1
  Sss28/1 -> Sum318/2
  Sum290/1 -> Mux47/1
  Demux31/2 -> Scope151/6, Sum177/1  "-30% F_PU"
  Sum307/1 -> Mux27/1
  Gain174/1 -> Sum174/1
  Gain177/1 -> Scope132/1
  Mux27/1 -> MATLAB Function27/1(u)  "u"
  Gain175/1 -> Sum175/1
  Sum178/1 -> Gain178/1
  Demux31/1 -> Sum176/1
  Gain311/1 -> Sum311/1
  Sum299/1 -> Gain299/1
  Gain267/1 -> Sum267/1
  Integrator28/1 -> MATLAB Function28/2(x), Demux28/1  "x"
  Constant104/1 -> Gain329/1
  Step30/1 -> Gain332/1
  Bss43/1 -> Sum272/2
  F0ss30/1 -> Sum332/2
  Demux46/2 -> Scope151/7, Sum172/1  "-30% Fc"
  Gain176/1 -> Scope131/1
  Gain316/1 -> Sum316/1
  Mux46/1 -> MATLAB Function46/1(u)  "u"
  Mux47/1 -> MATLAB Function47/1(u)  "u"
  F_PUss42/1 -> Sum260/2
  Xss30/1 -> Sum333/2
  Sum183/1 -> Mux47/2
  Sum323/1 -> Mux29/1
  Demux28/1 -> Sum317/1
  Constant96/1 -> Gain311/1
  Constant88/1 -> Gain280/1
  Constant78/1 -> Gain257/1
  Sum280/1 -> Mux45/4
  Step45/1 -> Gain282/1
  Constant112/1 -> Gain290/1
  Constant101/1 -> Gain331/1
  Demux26/1 -> Sum299/1
  Xss28/1 -> Sum317/2
  Sum327/1 -> Gain327/1
  Sss27/1 -> Sum309/2
  Gain302/1 -> Scope104/1
  Gain308/1 -> Scope106/1
  Sss31/1 -> Sum177/2
  Gain305/1 -> Sum305/1
  Demux29/1 -> Sum324/1
  Gain317/1 -> Scope116/1
  Gain319/1 -> Scope118/1
  Constant93/1 -> Gain307/1
  Sum171/1 -> Mux31/4
  F_PUss28/1 -> Sum315/2
  Constant90/1 -> Gain301/1
  Constant97/1 -> Gain316/1
  Constant126/1 -> Gain216/1
  Xss47/1 -> Sum291/2
  Sum311/1 -> Mux28/4
  Sum335/1 -> Gain335/1
  Gain330/1 -> Sum330/1
  Sum328/1 -> Gain328/1
  Sum317/1 -> Gain317/1
  S0ss27/1 -> Sum304/2
  Integrator26/1 -> MATLAB Function26/2(x), Demux26/1  "x"
  Constant103/1 -> Gain330/1
  Sum244/1 -> Mux33/2
  Step39/1 -> Gain228/1
  S0ss25/1 -> Sum303/2
  Sss34/1 -> Sum196/2
  Gain222/1 -> Scope10/1
  Sum199/1 -> Mux35/4
  Sum198/1 -> Gain198/1
  Demux32/1 -> Sum221/1
  Gain281/1 -> Scope5/1
  F_css40/1 -> Sum234/2
  Xss34/1 -> Sum195/2
  Step26/1 -> Gain297/1
  Xss24/1 -> Sum270/2
  F0ss34/1 -> Sum194/2
  Sum212/1 -> Gain212/1
  Gain180/1 -> Sum180/1
  Mux32/1 -> MATLAB Function32/1(u)  "u"
  Gain190/1 -> Sum190/1
  Bss47/1 -> Sum294/2
  Constant94/1 -> Gain315/1
  Gain335/1 -> Scope129/1
  Gain205/1 -> Scope144/1
  Sum205/1 -> Gain205/1
  Gain231/1 -> Scope24/1
  Sum215/1 -> Gain215/1
  Gain182/1 -> Sum182/1
  Mux31/1 -> MATLAB Function31/1(u)  "u"
  Sum285/1 -> Gain285/1
  Gain178/1 -> Scope133/1
  Gain198/1 -> Scope142/1
  F_css28/1 -> Sum312/2
  Constant89/1 -> Gain284/1
  Gain284/1 -> Sum284/1
  Mux45/1 -> MATLAB Function45/1(u)  "u"
  Gain282/1 -> Sum282/1
  Sum284/1 -> Mux45/1
  Sum286/1 -> Gain286/1
  Sum287/1 -> Gain287/1
  Gain257/1 -> Sum257/1
  F0ss29/1 -> Sum323/2
  Sum258/1 -> Mux42/3
  Gain273/1 -> Sum273/1
  S0ss44/1 -> Sum273/2
  MATLAB Function45/1(dxdt) -> Integrator45/1  "dxdt"
  Gain279/1 -> Scope81/1
  Gain251/1 -> Sum251/1
  F_PUss44/1 -> Sum275/2
  Gain288/1 -> Sum288/1
  Gain263/1 -> Scope63/1
  F_css44/1 -> Sum274/2
  Sum279/1 -> Gain279/1
  Sss26/1 -> Sum300/2
  Gain278/1 -> Scope77/1
  Constant83/1 -> Gain275/1
  Demux44/2 -> Sum278/1
  Demux44/3 -> Sum279/1
  Sum276/1 -> Mux44/1
  Sum175/1 -> Mux31/1
  S0ss43/1 -> Sum265/2
  Sum272/1 -> Gain272/1
  Sum177/1 -> Gain177/1
  Gain272/1 -> Scope74/1
  Sum269/1 -> Gain269/1
  MATLAB Function34/1(dxdt) -> Integrator34/1  "dxdt"
  F_css43/1 -> Sum266/2
  Sum267/1 -> Mux43/2
  Constant80/1 -> Gain267/1
  MATLAB Function43/1(dxdt) -> Integrator43/1  "dxdt"
  Gain271/1 -> Scope70/1
  Sum304/1 -> Mux27/4
  Gain191/1 -> Sum191/1
  F_PUss43/1 -> Sum267/2
  Sum257/1 -> Mux42/4
  F_css41/1 -> Sum251/2
  MATLAB Function42/1(dxdt) -> Integrator42/1  "dxdt"
  Sss42/1 -> Sum263/2
  Gain262/1 -> Scope59/1
  Gain260/1 -> Sum260/1
  Integrator42/1 -> MATLAB Function42/2(x), Demux42/1  "x"
  Sum264/1 -> Gain264/1
  Demux41/1 -> Scope152/4, Sum254/1  "+30% S0"
  Sum254/1 -> Gain254/1
  Gain328/1 -> Scope125/1
  S0ss41/1 -> Sum250/2
  Sum252/1 -> Mux41/2
  Sum321/1 -> Mux29/3
  Constant76/1 -> Gain253/1
  Gain275/1 -> Sum275/1
  Xss42/1 -> Sum262/2
  MATLAB Function47/1(dxdt) -> Integrator47/1  "dxdt"
  F_PUss41/1 -> Sum252/2
  Bss36/1 -> Sum249/2
  Sss40/1 -> Sum239/2
  Constant144/1 -> Gain245/1
  Sum245/1 -> Mux36/1
  Constant125/1 -> Gain217/1
  MATLAB Function41/1(dxdt) -> Integrator41/1  "dxdt"
  Gain249/1 -> Scope47/1
  Gain215/1 -> Scope149/1
  Gain246/1 -> Scope25/1
  Gain255/1 -> Scope52/1
  Demux36/1 -> Scope152/3, Sum246/1  "+30% Fc"
  Sum322/1 -> Mux29/2
  F0ss25/1 -> Sum170/2
  Gain247/1 -> Scope39/1
  Demux36/3 -> Sum249/1
  Sum247/1 -> Gain247/1
  Sss25/1 -> Sum192/2
  Sum260/1 -> Mux42/2
  Xss25/1 -> Sum181/2
  Gain265/1 -> Sum265/1
  Gain334/1 -> Scope128/1
  Constant128/1 -> Gain170/1
  Sum314/1 -> Mux25/3
  Demux46/1 -> Sum326/1
  Sum170/1 -> Mux25/1
  Gain169/1 -> Sum169/1
  Demux34/2 -> Sum196/1
  Constant106/1 -> Gain259/1
  Gain213/1 -> Scope148/1
  F0ss24/1 -> Sum259/2
  Demux24/1 -> Scope152/7, Sum270/1  "-30% Fc"
  Sum259/1 -> Mux24/1
  Gain270/1 -> Scope4/1
  Gain268/1 -> Sum268/1
  Sum168/1 -> Mux24/4
  Sum237/1 -> Mux40/1
  Demux25/2 -> Sum192/1
  F_PUss47/1 -> Sum183/2
  Sum310/1 -> Gain310/1
  Demux25/3 -> Sum203/1
  Sum331/1 -> Mux30/2
  Gain301/1 -> Sum301/1
  F0ss27/1 -> Sum307/2
  Gain326/1 -> Scope93/1
  Gain309/1 -> Scope110/1
  F_PUss29/1 -> Sum322/2
  Integrator27/1 -> MATLAB Function27/2(x), Demux27/1  "x"
  Gain323/1 -> Sum323/1
  Integrator46/1 -> MATLAB Function46/2(x), Demux46/1  "x"
  Sss24/1 -> Sum281/2
  Integrator31/1 -> MATLAB Function31/2(x), Demux31/1  "x"
  Sum239/1 -> Gain239/1
  S0ss26/1 -> Sum295/2
  Sss45/1 -> Sum286/2
  Demux45/3 -> Sum287/1
  Step36/1 -> Gain236/1
  Gain173/1 -> Sum173/1
  Sss30/1 -> Sum334/2
  Gain331/1 -> Sum331/1
  Xss26/1 -> Sum299/2
  Gain171/1 -> Sum171/1
  Sum330/1 -> Mux30/3
  Sum295/1 -> Mux26/4
  Sum293/1 -> Gain293/1
  F0ss44/1 -> Sum276/2
  Demux47/3 -> Sum294/1
  Sum308/1 -> Gain308/1
  MATLAB Function30/1(dxdt) -> Integrator30/1  "dxdt"
  Constant110/1 -> Gain313/1
  Gain303/1 -> Sum303/1
  Sum265/1 -> Mux43/4
  Step29/1 -> Gain323/1
  Sum207/1 -> Mux37/4
  Mux25/1 -> MATLAB Function25/1(u)  "u"
  Constant130/1 -> Gain226/1
  S0ss35/1 -> Sum199/2
  F_css32/1 -> Sum185/2
  MATLAB Function24/1(dxdt) -> Integrator24/1  "dxdt"
  F_css46/1 -> Sum289/2
  Gain218/1 -> Sum218/1
  S0ss28/1 -> Sum311/2
  Constant117/1 -> Gain314/1
  Gain212/1 -> Scope147/1
  Sss37/1 -> Sum213/2
  Sum263/1 -> Gain263/1
  Sum220/1 -> Gain220/1
  Integrator43/1 -> MATLAB Function43/2(x), Demux43/1  "x"
  F0ss32/1 -> Sum209/2
  Integrator37/1 -> MATLAB Function37/2(x), Demux37/1  "x"
  Demux26/3 -> Sum302/1
  F0ss39/1 -> Sum228/2
  Gain300/1 -> Scope100/1
  F0ss42/1 -> Sum261/2
  F_css37/1 -> Sum208/2
  Bss35/1 -> Sum206/2
  Sss38/1 -> Sum222/2
  Gain170/1 -> Sum170/1
  Mux35/1 -> MATLAB Function35/1(u)  "u"
  Sum228/1 -> Mux39/1
  Xss40/1 -> Sum238/2
  Gain207/1 -> Sum207/1
  Sum234/1 -> Mux40/3
  Sum270/1 -> Gain270/1
  Sum303/1 -> Mux25/4
  Constant140/1 -> Gain190/1
  F0ss41/1 -> Sum253/2
  Constant139/1 -> Gain214/1
  Sum281/1 -> Gain281/1
  Sss33/1 -> Sum188/2
  S0ss39/1 -> Sum224/2
  Gain238/1 -> Scope29/1
  Demux39/1 -> Sum229/1
  Constant102/1 -> Gain289/1
  Sum214/1 -> Mux36/4
  Demux39/2 -> Sum230/1
  Constant81/1 -> Gain266/1
  Xss37/1 -> Sum212/2
  MATLAB Function37/1(dxdt) -> Integrator37/1  "dxdt"
  Mux34/1 -> MATLAB Function34/1(u)  "u"
  Mux40/1 -> MATLAB Function40/1(u)  "u"
  Constant133/1 -> Gain232/1
  Mux37/1 -> MATLAB Function37/1(u)  "u"
  Sum169/1 -> Mux24/3
  Gain206/1 -> Scope145/1
  Constant113/1 -> Gain295/1
  Gain315/1 -> Sum315/1
  Step37/1 -> Gain208/1
  Sum288/1 -> Mux46/4
  Sum195/1 -> Gain195/1
  F_css42/1 -> Sum258/2
  Integrator45/1 -> MATLAB Function45/2(x), Demux45/1  "x"
  Demux34/3 -> Scope150/3, Sum198/1  "+30% Fc"
  Integrator32/1 -> MATLAB Function32/2(x), Demux32/1  "x"
  S0ss33/1 -> Sum242/2
  Sss41/1 -> Sum255/2
  Sum274/1 -> Mux44/3
  Sum225/1 -> Mux36/3
  Demux35/2 -> Sum205/1
  Gain189/1 -> Scope43/1
  MATLAB Function35/1(dxdt) -> Integrator35/1  "dxdt"
  Bss27/1 -> Sum310/2
  F_PUss31/1 -> Sum174/2
  Sum309/1 -> Gain309/1
  MATLAB Function46/1(dxdt) -> Integrator46/1  "dxdt"
  Integrator34/1 -> MATLAB Function34/2(x), Demux34/1  "x"
  S0ss31/1 -> Sum171/2
  Sum196/1 -> Gain196/1
  Gain172/1 -> Scope95/1
  Sum202/1 -> Mux35/1
  Sum249/1 -> Gain249/1
  Sum188/1 -> Gain188/1
  Sum300/1 -> Gain300/1
  MATLAB Function31/1(dxdt) -> Integrator31/1  "dxdt"
  Step28/1 -> Gain312/1
  Demux30/3 -> Sum335/1
  Sum277/1 -> Gain277/1
  Gain298/1 -> Sum298/1
  F0ss28/1 -> Sum316/2
  F_css26/1 -> Sum296/2
  Xss41/1 -> Sum254/2
  Step24/1 -> Gain168/1
  Constant131/1 -> Gain224/1
  F_css31/1 -> Sum173/2
  Bss46/1 -> Sum179/2
  Sum187/1 -> Gain187/1
  Step44/1 -> Gain276/1
  Constant92/1 -> Gain305/1
  Bss29/1 -> Sum328/2
  Sum229/1 -> Gain229/1
  Step34/1 -> Gain193/1
  Sum235/1 -> Mux40/2
  Gain243/1 -> Sum243/1
  Gain250/1 -> Sum250/1
  Constant116/1 -> Gain197/1
  Sum305/1 -> Mux27/3
  Sum332/1 -> Mux30/1
  Mux29/1 -> MATLAB Function29/1(u)  "u"
  Gain184/1 -> Sum184/1
  Sum201/1 -> Mux35/2
  Gain329/1 -> Sum329/1
  Gain325/1 -> Sum325/1
  Constant142/1 -> Gain194/1
  Demux27/1 -> Sum308/1
  Xss29/1 -> Sum324/2
  Sum243/1 -> Mux33/3
  MATLAB Function27/1(dxdt) -> Integrator27/1  "dxdt"
  Xss35/1 -> Sum204/2
  F_css45/1 -> Sum282/2
  Sum291/1 -> Gain291/1
  Xss46/1 -> Sum326/2
  F0ss40/1 -> Sum237/2
  Gain289/1 -> Sum289/1
  Demux38/2 -> Sum222/1
  Gain277/1 -> Scope76/1
  F_css33/1 -> Sum243/2
  Gain225/1 -> Sum225/1
  Constant99/1 -> Gain321/1
  Constant109/1 -> Gain183/1
  Gain197/1 -> Sum197/1
  Gain258/1 -> Sum258/1
  Integrator44/1 -> MATLAB Function44/2(x), Demux44/1  "x"
  MATLAB Function40/1(dxdt) -> Integrator40/1  "dxdt"
  F_PUss36/1 -> Sum236/2
  Sum193/1 -> Mux34/2
  Constant137/1 -> Gain243/1
  Demux42/3 -> Sum264/1
  Gain237/1 -> Sum237/1
  Bss45/1 -> Sum287/2
  Gain229/1 -> Scope19/1
  S0ss29/1 -> Sum320/2
  Constant114/1 -> Gain296/1
  Mux33/1 -> MATLAB Function33/1(u)  "u"
  Gain280/1 -> Sum280/1
  Gain248/1 -> Sum248/1
  Sum312/1 -> Mux28/3
  Bss40/1 -> Sum240/2
  Mux42/1 -> MATLAB Function42/1(u)  "u"
  Sss43/1 -> Sum271/2
  Step42/1 -> Gain258/1
  Sum180/1 -> Mux47/4
  Sum174/1 -> Mux31/2
  Demux32/3 -> Scope150/7, Sum241/1  "-30% Fc"
  Sss46/1 -> Sum172/2
  Sum255/1 -> Gain255/1
  F_css27/1 -> Sum305/2
  Demux44/1 -> Scope152/2, Sum277/1  "+30% F_PU"
  Xss27/1 -> Sum308/2
  Gain320/1 -> Sum320/1
  Sum204/1 -> Gain204/1
  Constant74/1 -> Gain250/1
  F0ss47/1 -> Sum290/2
  Integrator38/1 -> MATLAB Function38/2(x), Demux38/1  "x"
  Gain203/1 -> Scope136/1
  Step27/1 -> Gain306/1
  MATLAB Function36/1(dxdt) -> Integrator36/1  "dxdt"
  Bss42/1 -> Sum264/2
  Sum273/1 -> Mux44/4
  Sum262/1 -> Gain262/1
  Demux46/3 -> Sum179/1
  F_css25/1 -> Sum314/2
  Constant86/1 -> Gain273/1
  Step43/1 -> Gain268/1
  F_PUss30/1 -> Sum331/2
  Sss47/1 -> Sum293/2
  Gain195/1 -> Scope140/1
  Sum294/1 -> Gain294/1
  Xss36/1 -> Sum246/2
  Gain297/1 -> Sum297/1
  MATLAB Function29/1(dxdt) -> Integrator29/1  "dxdt"
  Constant123/1 -> Gain211/1
  Gain310/1 -> Scope111/1
  Gain235/1 -> Sum235/1
  Sum289/1 -> Mux46/3
  Sum334/1 -> Gain334/1
  Mux41/1 -> MATLAB Function41/1(u)  "u"
  Sum250/1 -> Mux41/4
  Sum282/1 -> Mux45/3
  F_css35/1 -> Sum200/2
  Gain224/1 -> Sum224/1
  Demux30/1 -> Sum333/1
  Gain228/1 -> Sum228/1
  Sum301/1 -> Mux46/2
  Bss31/1 -> Sum178/2
  Constant107/1 -> Gain171/1
  Sum271/1 -> Gain271/1
  Step31/1 -> Gain173/1
  Gain239/1 -> Scope30/1
  Gain299/1 -> Scope99/1
  Demux31/3 -> Sum178/1
  Sum275/1 -> Mux44/2
  Demux28/2 -> Scope151/5, Sum318/1  "-30% F0"
  Mux24/1 -> MATLAB Function24/1(u)  "u"
  Constant77/1 -> Gain260/1
  Sum231/1 -> Gain231/1
  Sum213/1 -> Gain213/1
  Sum329/1 -> Mux30/4
  F_PUss32/1 -> Sum197/2
  Constant120/1 -> Gain202/1
  Sum238/1 -> Gain238/1
  Sum216/1 -> Mux38/4
  S0ss38/1 -> Sum216/2
  Bss26/1 -> Sum302/2
  Sum315/1 -> Mux28/2
  Sum208/1 -> Mux37/3
  F_css34/1 -> Sum191/2
  Gain245/1 -> Sum245/1
  F_css47/1 -> Sum182/2
  Step32/1 -> Gain184/1
  F0ss38/1 -> Sum219/2
  MATLAB Function44/1(dxdt) -> Integrator44/1  "dxdt"
  Sum172/1 -> Gain172/1
  Sum241/1 -> Gain241/1
  Sum261/1 -> Mux42/1
  Step38/1 -> Gain219/1
  Gain293/1 -> Scope135/1
  Bss33/1 -> Sum189/2
  Sum192/1 -> Gain192/1
  Gain269/1 -> Scope69/1
  Gain193/1 -> Sum193/1
  MATLAB Function28/1(dxdt) -> Integrator28/1  "dxdt"
  Demux39/3 -> Scope150/2, Sum231/1  "+30% F_PU"
  Bss28/1 -> Sum319/2
  F_PUss25/1 -> Sum325/2
  S0ss30/1 -> Sum329/2
  Sss44/1 -> Sum278/2
  Sum221/1 -> Gain221/1
  Demux25/1 -> Scope152/8, Sum181/1  "-30% S0"
  Sum298/1 -> Mux26/1
  Constant84/1 -> Gain169/1
  Sum251/1 -> Mux41/3
  F0ss45/1 -> Sum284/2
  Gain232/1 -> Sum232/1
  Constant122/1 -> Gain207/1
  Xss43/1 -> Sum269/2
  Sum278/1 -> Gain278/1
  Demux24/2 -> Sum281/1
  Gain291/1 -> Scope134/1
  Sum236/1 -> Mux36/2
  Demux26/2 -> Scope151/3, Sum300/1  "+30% Fc"
  Sum319/1 -> Gain319/1
  Sum296/1 -> Mux26/3
  Gain200/1 -> Sum200/1
  Gain186/1 -> Sum186/1
  Constant135/1 -> Gain244/1
  MATLAB Function32/1(dxdt) -> Integrator32/1  "dxdt"
  Integrator39/1 -> MATLAB Function39/2(x), Demux39/1  "x"
  Sum326/1 -> Gain326/1
  F0ss31/1 -> Sum175/2
  Constant100/1 -> Gain320/1
  Demux24/3 -> Sum292/1
  Gain306/1 -> Sum306/1
  Gain208/1 -> Sum208/1
  Sum176/1 -> Gain176/1
  Demux33/1 -> Sum187/1
  Demux34/1 -> Sum195/1
  Gain185/1 -> Sum185/1
  Bss24/1 -> Sum292/2
  Demux45/2 -> Sum286/1
  Step46/1 -> Gain288/1
  Gain214/1 -> Sum214/1
  Gain236/1 -> Sum236/1
  Gain220/1 -> Scope9/1
  Step35/1 -> Gain201/1
  Gain199/1 -> Sum199/1
  S0ss24/1 -> Sum168/2
  Gain226/1 -> Sum226/1
  Integrator29/1 -> MATLAB Function29/2(x), Demux29/1  "x"
  Gain201/1 -> Sum201/1
  Sum253/1 -> Mux41/1
  Mux44/1 -> MATLAB Function44/1(u)  "u"
  Demux28/3 -> Sum319/1
  Gain313/1 -> Sum313/1
  S0ss45/1 -> Sum280/2
  Demux42/1 -> Scope152/5, Sum262/1  "-30% F0"
  Bss25/1 -> Sum203/2
  Step33/1 -> Gain242/1
  Sum227/1 -> Mux39/2
  Constant75/1 -> Gain251/1
  MATLAB Function26/1(dxdt) -> Integrator26/1  "dxdt"
  Xss32/1 -> Sum221/2
  Mux39/1 -> MATLAB Function39/1(u)  "u"
  Gain183/1 -> Sum183/1
  Integrator35/1 -> MATLAB Function35/2(x), Demux35/1  "x"
  Gain194/1 -> Sum194/1
  Gain227/1 -> Sum227/1
  Gain202/1 -> Sum202/1
  Sss32/1 -> Sum233/2
  Gain241/1 -> Scope146/1
  Sum313/1 -> Mux46/1
  Gain188/1 -> Scope40/1
  Bss32/1 -> Sum241/2
  Sum248/1 -> Mux24/2
  Constant129/1 -> Gain185/1
  S0ss46/1 -> Sum288/2
  Sum191/1 -> Mux34/3
  Xss45/1 -> Sum285/2
  Sum203/1 -> Gain203/1
  Gain292/1 -> Scope58/1
  F_PUss34/1 -> Sum193/2
  F_PUss27/1 -> Sum306/2
  F0ss35/1 -> Sum202/2
  Demux43/3 -> Sum272/1
  Xss31/1 -> Sum176/2
  Sum232/1 -> Mux40/4
  F_css38/1 -> Sum217/2
  Gain242/1 -> Sum242/1
  S0ss34/1 -> Sum190/2
  Sum318/1 -> Gain318/1
  Gain266/1 -> Sum266/1
  Bss38/1 -> Sum223/2
  MATLAB Function33/1(dxdt) -> Integrator33/1  "dxdt"
  Integrator30/1 -> MATLAB Function30/2(x), Demux30/1  "x"
  Sum240/1 -> Gain240/1
  Sum306/1 -> Mux27/2
  Sum316/1 -> Mux28/1
  Demux37/1 -> Sum212/1
  Step40/1 -> Gain234/1
  Demux41/3 -> Sum256/1
  Sum182/1 -> Mux47/3
  Sum302/1 -> Gain302/1
  Demux40/1 -> Sum238/1
  Constant73/1 -> Gain248/1
  Mux26/1 -> MATLAB Function26/1(u)  "u"
  Sum325/1 -> Mux25/2
  Constant132/1 -> Gain235/1
  Gain219/1 -> Sum219/1
  Constant87/1 -> Gain283/1
  Gain168/1 -> Sum168/1
  Gain283/1 -> Sum283/1
  Sum320/1 -> Mux29/4
  Sum242/1 -> Mux33/4
  Gain244/1 -> Sum244/1
  Sum233/1 -> Gain233/1
  Sum186/1 -> Mux33/1
  Gain295/1 -> Sum295/1
  Integrator25/1 -> MATLAB Function25/2(x), Demux25/1  "x"
  Constant119/1 -> Gain200/1
  Sum292/1 -> Gain292/1
  Mux43/1 -> MATLAB Function43/1(u)  "u"
  Gain192/1 -> Scope130/1
  Xss39/1 -> Sum229/2
  Demux36/2 -> Sum247/1
  Demux47/2 -> Scope151/8, Sum293/1  "-30% S0"
  Integrator33/1 -> MATLAB Function33/2(x), Demux33/1  "x"
  Gain221/1 -> Scope138/1
  S0ss47/1 -> Sum180/2
  Constant143/1 -> Gain225/1
  Integrator41/1 -> MATLAB Function41/2(x), Demux41/1  "x"
  Constant127/1 -> Gain227/1
  Sum197/1 -> Mux32/2
  Sum218/1 -> Mux38/2
  Sss39/1 -> Sum230/2
  Demux42/2 -> Sum263/1
  Sss36/1 -> Sum247/2
  Sum200/1 -> Mux35/3
  Demux27/2 -> Scope151/4, Sum309/1  "+30% S0"
  Gain264/1 -> Scope65/1
  Constant98/1 -> Gain322/1
  Sum217/1 -> Mux38/3
  Mux30/1 -> MATLAB Function30/1(u)  "u"
  Constant111/1 -> Gain182/1
  Bss44/1 -> Sum279/2
  Gain287/1 -> Scope89/1
  F0ss37/1 -> Sum211/2
  Gain307/1 -> Sum307/1
  Sss29/1 -> Sum327/2
  Demux38/3 -> Scope150/1, Sum223/1  "+30% F0"
  Constant134/1 -> Gain237/1
  F_PUss38/1 -> Sum218/2
  Sum246/1 -> Gain246/1
  MATLAB Function25/1(dxdt) -> Integrator25/1  "dxdt"
  Mux28/1 -> MATLAB Function28/1(u)  "u"
  S0ss37/1 -> Sum207/2
  F0ss36/1 -> Sum245/2
  Demux43/2 -> Sum271/1
  Gain332/1 -> Sum332/1
  Sum209/1 -> Mux32/1
  S0ss40/1 -> Sum232/2
  F_PUss35/1 -> Sum201/2
  Gain179/1 -> Scope115/1
  Sum210/1 -> Mux37/2
  Gain233/1 -> Scope139/1
  Demux40/3 -> Scope150/6, Sum240/1  "-30% F_PU"
  Gain274/1 -> Sum274/1
  Gain259/1 -> Sum259/1
  Demux35/3 -> Scope150/4, Sum206/1  "+30% S0"
  Constant118/1 -> Gain199/1
  Gain296/1 -> Sum296/1
  Integrator36/1 -> MATLAB Function36/2(x), Demux36/1  "x"
  F_PUss39/1 -> Sum227/2
  Constant141/1 -> Gain191/1
  Gain216/1 -> Sum216/1
  Gain286/1 -> Scope88/1
  Demux30/2 -> Scope151/2, Sum334/1  "+30% F_PU"
  F0ss46/1 -> Sum313/2
  Step47/1 -> Gain180/1
  F_css29/1 -> Sum321/2
  Xss38/1 -> Sum220/2
  Sum185/1 -> Mux32/3
  Constant91/1 -> Gain304/1
  Gain321/1 -> Sum321/1
  Integrator40/1 -> MATLAB Function40/2(x), Demux40/1  "x"
  Sum181/1 -> Gain181/1
  Constant124/1 -> Gain218/1
  Constant121/1 -> Gain210/1
  Demux29/2 -> Scope151/1, Sum327/1  "+30% F0"
  Xss44/1 -> Sum277/2
  Gain240/1 -> Scope34/1
  F_PUss24/1 -> Sum248/2
  Constant79/1 -> Gain261/1
  Demux32/2 -> Sum233/1
  Demux45/1 -> Scope152/6, Sum285/1  "-30% F_PU"
  F_css36/1 -> Sum225/2
  F0ss33/1 -> Sum186/2
  Sum222/1 -> Gain222/1
  Mux36/1 -> MATLAB Function36/1(u)  "u"
  Gain254/1 -> Scope48/1
  Sum179/1 -> Gain179/1
  Constant95/1 -> Gain325/1
  Mux38/1 -> MATLAB Function38/1(u)  "u"
  Gain304/1 -> Sum304/1
  Gain252/1 -> Sum252/1
  Demux40/2 -> Sum239/1
  Sum190/1 -> Mux34/4
  Sum324/1 -> Gain324/1
  Gain181/1 -> Scope122/1
  Sum266/1 -> Mux43/3
  Gain318/1 -> Scope117/1
  Sum256/1 -> Gain256/1
  Demux37/2 -> Sum213/1
  Gain204/1 -> Scope143/1
  Gain322/1 -> Sum322/1
  Sum211/1 -> Mux37/1
  Constant105/1 -> Gain174/1
  F_css39/1 -> Sum226/2
  Sum206/1 -> Gain206/1
  Bss41/1 -> Sum256/2
  Gain217/1 -> Sum217/1
  Sum194/1 -> Mux34/1
  Gain256/1 -> Scope54/1
  Step25/1 -> Gain303/1
  Gain234/1 -> Sum234/1
  Constant82/1 -> Gain265/1
  F_PUss45/1 -> Sum283/2
  Gain285/1 -> Scope84/1
  Demux43/1 -> Scope152/1, Sum269/1  "+30% F0"
  Sum189/1 -> Gain189/1
  Constant85/1 -> Gain274/1
  Gain211/1 -> Sum211/1
  Bss39/1 -> Sum231/2
  Gain312/1 -> Sum312/1
  S0ss42/1 -> Sum257/2
  F_PUss26/1 -> Sum297/2
  Demux27/3 -> Sum310/1
  F0ss26/1 -> Sum298/2
  Demux33/3 -> Scope150/8, Sum189/1  "-30% S0"
  Sum219/1 -> Mux38/1
  Constant108/1 -> Gain175/1
  Gain223/1 -> Scope14/1
  Sum297/1 -> Mux26/2
  F_css30/1 -> Sum330/2
  Constant115/1 -> Gain298/1
  Gain290/1 -> Sum290/1
  F_PUss40/1 -> Sum235/2
  Step41/1 -> Gain252/1
  Constant136/1 -> Gain209/1
  Gain261/1 -> Sum261/1
  Sum268/1 -> Mux43/1
  F0ss43/1 -> Sum268/2
  Gain314/1 -> Sum314/1
  S0ss36/1 -> Sum214/2
  Bss34/1 -> Sum198/2
  Sum226/1 -> Mux39/3
  Integrator24/1 -> MATLAB Function24/2(x), Demux24/1  "x"
  Gain209/1 -> Sum209/1
  F_PUss46/1 -> Sum301/2
  Demux29/3 -> Sum328/1
  Gain196/1 -> Scope141/1
  Gain276/1 -> Sum276/1
  Sum283/1 -> Mux45/2
  Gain333/1 -> Scope127/1
  Sum184/1 -> Mux32/4
  S0ss32/1 -> Sum184/2
  Demux47/1 -> Sum291/1
  Gain327/1 -> Scope124/1
  F_PUss33/1 -> Sum244/2
  Gain230/1 -> Scope20/1
  Bss30/1 -> Sum335/2
  Gain294/1 -> Scope137/1
  Gain253/1 -> Sum253/1
